simulink model "Shaddad_BMS"  (R2026b)
undefined symbols (not defined in the file): CAN, FD, P, Ts
libraries: simulink x39, stm32blockslib x12, BatteryProtection x7, dspstat3 x7, BatteryEstimators x4, BatteryCurrentManagement x3, eeGeneralControl x2, BatteryBalancing x1, BatterySoeEstimators x1, BatteryPowerEstimators x1, BatteryThermalManagement x1, svdutilitieslib x1
(part 2 of 2)

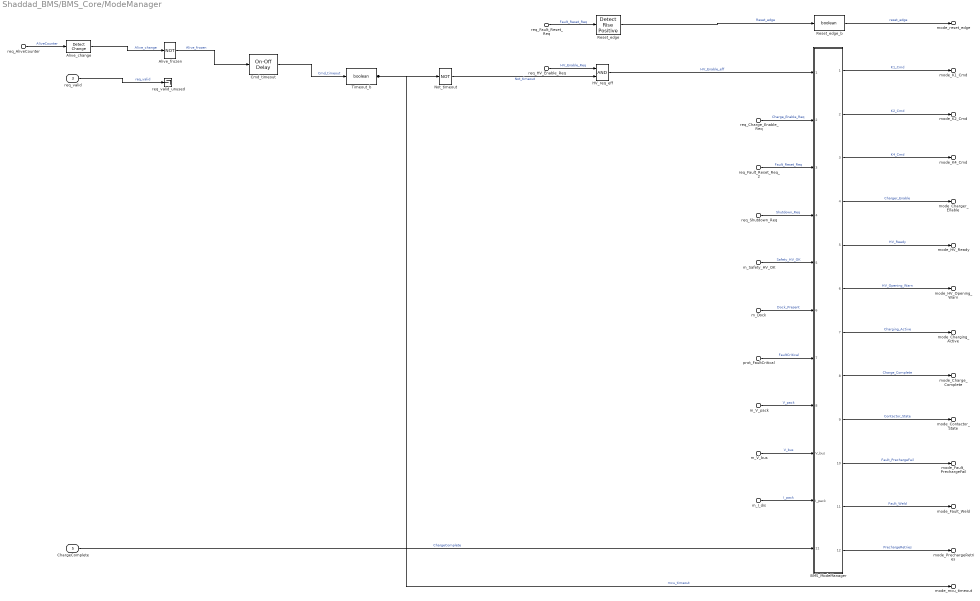
== system Shaddad_BMS/BMS_Core/ModeManager ==
  m_Safety_HV_OK : Inport  PortName=m  Element=Safety_HV_OK
  m_Dock : Inport  PortName=m  Element=Dock
  m_V_pack : Inport  PortName=m  Element=V_pack
  m_V_bus : Inport  PortName=m  Element=V_bus
  m_I_dis : Inport  PortName=m  Element=I_dis
  req_AliveCounter : Inport  Port=2  PortName=req  Element=AliveCounter
  req_HV_Enable_Req : Inport  Port=2  PortName=req  Element=HV_Enable_Req
  req_Fault_Reset_Req : Inport  Port=2  PortName=req  Element=Fault_Reset_Req
  req_Fault_Reset_Req_2 : Inport  Port=2  PortName=req  Element=Fault_Reset_Req
  req_Charge_Enable_Req : Inport  Port=2  PortName=req  Element=Charge_Enable_Req
  req_Shutdown_Req : Inport  Port=2  PortName=req  Element=Shutdown_Req
  req_valid : Inport  Port=3
  prot_FaultCritical : Inport  Port=4  PortName=prot  Element=FaultCritical
  ChargeComplete : Inport  Port=5
  Alive_change : simulink/Logic and Bit Operations/Detect Change  vinit=0  OutDataTypeStr=boolean
  Alive_frozen : Logic  Operator=NOT  AllPortsSameDT=off  OutDataTypeStr=boolean
  BMS_ModeManager : MATLAB Function  TreatAsAtomicUnit=on  mask{prm=P.power.bms.chart}
      mask prompts: prm "Mode manager parameters"
  Cmd_timeout : eeGeneralControl/On-Off Delay  LabelModeActiveChoice=Discrete  Td_on=P.power.bms.mcu_cmd_timeout  Td_off=0  IC=0  Ts=Ts.bms_fast
      settings: LibrarySourceBlock=ee_sl_lib/General Control/On-Off Delay
  HV_req_eff : Logic  AllPortsSameDT=off  OutDataTypeStr=boolean
  Not_timeout : Logic  Operator=NOT  AllPortsSameDT=off  OutDataTypeStr=boolean
  Reset_edge : simulink/Logic and Bit Operations/Detect Rise Positive  vinit=0  OutDataTypeStr=boolean
  Reset_edge_b : DataTypeConversion  OutDataTypeStr=boolean  SaturateOnIntegerOverflow=off  RndMeth=Floor
  Timeout_b : DataTypeConversion  OutDataTypeStr=boolean  SaturateOnIntegerOverflow=off  RndMeth=Floor
  req_valid_unused : Terminator
  mode_mcu_timeout : Outport  PortName=mode  Element=mcu_timeout
  mode_reset_edge : Outport  PortName=mode  Element=reset_edge
  mode_K1_Cmd : Outport  PortName=mode  Element=K1_Cmd
  mode_K2_Cmd : Outport  PortName=mode  Element=K2_Cmd
  mode_K4_Cmd : Outport  PortName=mode  Element=K4_Cmd
  mode_Charger_Enable : Outport  PortName=mode  Element=Charger_Enable
  mode_HV_Ready : Outport  PortName=mode  Element=HV_Ready
  mode_HV_Opening_Warn : Outport  PortName=mode  Element=HV_Opening_Warn
  mode_Charging_Active : Outport  PortName=mode  Element=Charging_Active
  mode_Charge_Complete : Outport  PortName=mode  Element=Charge_Complete
  mode_Contactor_State : Outport  PortName=mode  Element=Contactor_State
  mode_Fault_PrechargeFail : Outport  PortName=mode  Element=Fault_PrechargeFail
  mode_Fault_Weld : Outport  PortName=mode  Element=Fault_Weld
  mode_PrechargeRetries : Outport  PortName=mode  Element=PrechargeRetries
  wires:
  req_AliveCounter/1 -> Alive_change/1  "AliveCounter"
  req_valid/1 -> req_valid_unused/1  "req_valid"
  ChargeComplete/1 -> BMS_ModeManager/11(ChargeComplete)  "ChargeComplete"
  Alive_change/1 -> Alive_frozen/1  "Alive_change"
  Alive_frozen/1 -> Cmd_timeout/1  "Alive_frozen"
  Cmd_timeout/1 -> Timeout_b/1  "Cmd_timeout"
  Timeout_b/1 -> mode_mcu_timeout/1, Not_timeout/1  "mcu_timeout"
  Not_timeout/1 -> HV_req_eff/2  "Not_timeout"
  req_Fault_Reset_Req/1 -> Reset_edge/1  "Fault_Reset_Req"
  req_HV_Enable_Req/1 -> HV_req_eff/1  "HV_Enable_Req"
  HV_req_eff/1 -> BMS_ModeManager/1(HV_Enable_Req)  "HV_Enable_eff"
  Reset_edge/1 -> Reset_edge_b/1  "Reset_edge"
  req_Charge_Enable_Req/1 -> BMS_ModeManager/2(Charge_Enable_Req)  "Charge_Enable_Req"
  req_Fault_Reset_Req_2/1 -> BMS_ModeManager/3(Fault_Reset_Req)  "Fault_Reset_Req"
  req_Shutdown_Req/1 -> BMS_ModeManager/4(Shutdown_Req)  "Shutdown_Req"
  m_Safety_HV_OK/1 -> BMS_ModeManager/5(Safety_OK)  "Safety_HV_OK"
  m_Dock/1 -> BMS_ModeManager/6(Dock_Present)  "Dock_Present"
  prot_FaultCritical/1 -> BMS_ModeManager/7(FaultCritical)  "FaultCritical"
  m_V_pack/1 -> BMS_ModeManager/8(V_pack)  "V_pack"
  m_V_bus/1 -> BMS_ModeManager/9(V_bus)  "V_bus"
  m_I_dis/1 -> BMS_ModeManager/10(I_pack)  "I_pack"
  BMS_ModeManager/1(K1_Cmd) -> mode_K1_Cmd/1  "K1_Cmd"
  BMS_ModeManager/2(K2_Cmd) -> mode_K2_Cmd/1  "K2_Cmd"
  BMS_ModeManager/3(K4_Cmd) -> mode_K4_Cmd/1  "K4_Cmd"
  BMS_ModeManager/4(Charger_Enable) -> mode_Charger_Enable/1  "Charger_Enable"
  BMS_ModeManager/5(HV_Ready) -> mode_HV_Ready/1  "HV_Ready"
  BMS_ModeManager/6(HV_Opening_Warn) -> mode_HV_Opening_Warn/1  "HV_Opening_Warn"
  BMS_ModeManager/7(Charging_Active) -> mode_Charging_Active/1  "Charging_Active"
  BMS_ModeManager/8(Charge_Complete) -> mode_Charge_Complete/1  "Charge_Complete"
  BMS_ModeManager/9(Contactor_State) -> mode_Contactor_State/1  "Contactor_State"
  BMS_ModeManager/10(Fault_PrechargeFail) -> mode_Fault_PrechargeFail/1  "Fault_PrechargeFail"
  BMS_ModeManager/11(Fault_Weld) -> mode_Fault_Weld/1  "Fault_Weld"
  BMS_ModeManager/12(PrechargeRetries) -> mode_PrechargeRetries/1  "PrechargeRetries"
  Reset_edge_b/1 -> mode_reset_edge/1  "reset_edge"

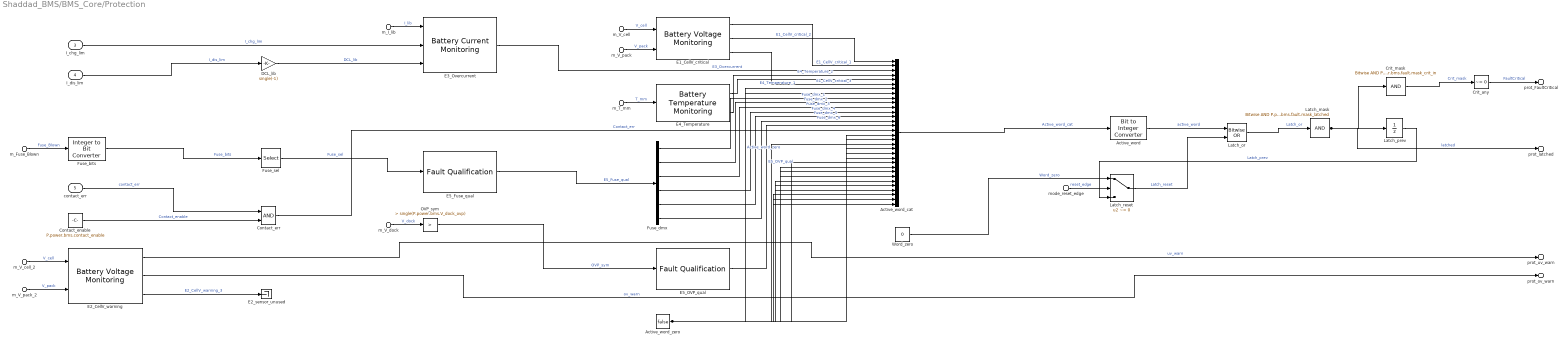
== system Shaddad_BMS/BMS_Core/Protection ==
  m_V_cell : Inport  PortName=m  Element=V_cell
  m_V_cell_2 : Inport  PortName=m  Element=V_cell
  m_V_pack : Inport  PortName=m  Element=V_pack
  m_V_pack_2 : Inport  PortName=m  Element=V_pack
  m_I_lib : Inport  PortName=m  Element=I_lib
  m_T_mm : Inport  PortName=m  Element=T_mm
  m_Fuse_Blown : Inport  PortName=m  Element=Fuse_Blown
  m_V_dock : Inport  PortName=m  Element=V_dock
  mode_reset_edge : Inport  Port=2  PortName=mode  Element=reset_edge
  I_chg_lim : Inport  Port=3
  I_dis_lim : Inport  Port=4
  contact_err : Inport  Port=5
  Active_word : simulink/Logic and Bit Operations/Bit to Integer Converter  nbits=32  bitOrder=LSB first  signedOutputValues=Unsigned  outDtype=uint32  outDtypeSigned=Inherit via internal rule
      settings: LibrarySourceBlock=|
      | commutil2/Bit to Integer
      | Converter
  Active_word_cat : Concatenate  NumInputs=32
  Active_word_zero : Constant  Value=false  OutDataTypeStr=boolean  SampleTime=Ts.bms_fast
  Contact_enable : Constant  Value=P.power.bms.contact_enable  OutDataTypeStr=boolean  SampleTime=Ts.bms_fast
  Contact_err : Logic  AllPortsSameDT=off  OutDataTypeStr=boolean
  Crit_any : simulink/Logic and Bit Operations/Compare To Zero  relop=~=  OutDataTypeStr=boolean
  Crit_mask : simulink/Logic and Bit Operations/Bitwise Operator  logicop=AND  UseBitMask=on  BitMask=P.power.bms.fault.mask_crit_in  BitMaskRealWorld=Stored Integer
  DCL_lib : Gain  Gain=single(-1)
  E1_CellV_critical : BatteryProtection/Battery Voltage Monitoring  UndervoltageLimit=single(P.power.bms.V_uv)  OvervoltageLimit=single(P.power.bms.V_ov)  FaultySensorThreshold=single(P.power.bms.FaultySensorThreshold)  QualTimeUndervoltage=P.power.bms.qual.UV  DisqualTimeUndervoltage=P.power.bms.disqual  QualTimeOvervoltage=P.power.bms.qual.OV  DisqualTimeOvervoltage=P.power.bms.disqual  QualTimeSensorFaulty=P.power.bms.qual.sensor  DisqualTimeSensorFaulty=P.power.bms.disqual  Ts=-1  DataType=single
      settings: LibrarySourceBlock=|
      | batt_sl_lib/Protection/Battery Voltage
      | Monitoring
  E2_CellV_warning : BatteryProtection/Battery Voltage Monitoring  UndervoltageLimit=single(P.power.bms.V_uv_warn)  OvervoltageLimit=single(P.power.bms.V_ov_warn)  FaultySensorThreshold=single(P.power.bms.FaultySensorThreshold)  QualTimeUndervoltage=5  DisqualTimeUndervoltage=5  QualTimeOvervoltage=5  DisqualTimeOvervoltage=5  QualTimeSensorFaulty=5  DisqualTimeSensorFaulty=5  Ts=-1  DataType=single
      settings: LibrarySourceBlock=|
      | batt_sl_lib/Protection/Battery Voltage
      | Monitoring
  E2_sensor_unused : Terminator
  E3_Overcurrent : BatteryProtection/Battery Current Monitoring  ErrorLimit=single(P.power.bms.OC_ErrorLimit)  QualTime=P.power.bms.qual.OC  DisqualTime=P.power.bms.disqual  Ts=-1  DataType=single
      settings: LibrarySourceBlock=|
      | batt_sl_lib/Protection/Battery Current
      | Monitoring
  E4_Temperature : BatteryProtection/Battery Temperature Monitoring  MinMaxFlag=on  UndertemperatureLimit=single(P.power.bms.T_ut)  OvertemperatureLimit=single(P.power.bms.T_ot)  QualTimeUndertemp=P.power.bms.qual.OT  DisqualTimeUndertemp=P.power.bms.disqual  QualTimeOvertemp=P.power.bms.qual.OT  DisqualTimeOvertemp=P.power.bms.disqual  Ts=-1  DataType=single
      settings: LibrarySourceBlock=|
      | batt_sl_lib/Protection/Battery Temperature
      | Monitoring
  E5_Fuse_qual : BatteryProtection/Fault Qualification  QualTime=P.power.bms.qual_aux  DisqualTime=P.power.bms.disqual  Ts=-1
      settings: LibrarySourceBlock=batt_sl_lib/Protection/Fault Qualification
  E5_OVP_qual : BatteryProtection/Fault Qualification  QualTime=P.power.bms.qual_aux  DisqualTime=P.power.bms.disqual  Ts=-1
      settings: LibrarySourceBlock=batt_sl_lib/Protection/Fault Qualification
  Fuse_bits : simulink/Logic and Bit Operations/Integer to Bit Converter  nbits=8  signedInputValues=Unsigned  bitOrder=LSB first  outDtype=boolean
      settings: LibrarySourceBlock=|
      | commutil2/Integer to Bit
      | Converter
  Fuse_dmx : Demux  Outputs=6
  Fuse_sel : Selector  InputPortWidth=8  IndexOptions=Index vector (dialog)  Indices=1:6  OutputSizes=1
  Latch_mask : simulink/Logic and Bit Operations/Bitwise Operator  logicop=AND  UseBitMask=on  BitMask=P.power.bms.fault.mask_latched  BitMaskRealWorld=Stored Integer
  Latch_or : simulink/Logic and Bit Operations/Bitwise Operator  logicop=OR  UseBitMask=off  NumInputPorts=2  BitMask=bin2dec('11011001')  BitMaskRealWorld=Stored Integer
  Latch_prev : UnitDelay  InitialCondition=uint32(0)  SampleTime=Ts.bms_fast
  Latch_reset : Switch  Criteria=u2 ~= 0  SaturateOnIntegerOverflow=off  InputSameDT=off
  OVP_sym : simulink/Logic and Bit Operations/Compare To Constant  relop=>  const=single(P.power.bms.V_dock_ovp)  OutDataTypeStr=boolean
  Word_zero : Constant  Value=0  OutDataTypeStr=uint32  SampleTime=Ts.bms_fast
  prot_uv_warn : Outport  PortName=prot  Element=uv_warn
  prot_ov_warn : Outport  PortName=prot  Element=ov_warn
  prot_latched : Outport  PortName=prot  Element=latched
  prot_FaultCritical : Outport  PortName=prot  Element=FaultCritical
  wires:
  m_Fuse_Blown/1 -> Fuse_bits/1  "Fuse_Blown"
  m_V_cell_2/1 -> E2_CellV_warning/1  "V_cell"
  m_V_pack_2/1 -> E2_CellV_warning/2  "V_pack"
  I_chg_lim/1 -> E3_Overcurrent/2  "I_chg_lim"
  I_dis_lim/1 -> DCL_lib/1  "I_dis_lim"
  contact_err/1 -> Contact_err/1  "contact_err"
  Contact_enable/1 -> Contact_err/2  "Contact_enable"
  Fuse_bits/1 -> Fuse_sel/1  "Fuse_bits"
  E2_CellV_warning/1 -> prot_uv_warn/1  "uv_warn"
  E2_CellV_warning/2 -> prot_ov_warn/1  "ov_warn"
  E2_CellV_warning/3 -> E2_sensor_unused/1  "E2_CellV_warning_3"
  DCL_lib/1 -> E3_Overcurrent/3  "DCL_lib"
  Contact_err/1 -> Active_word_cat/16  "Contact_err"
  Fuse_sel/1 -> E5_Fuse_qual/1  "Fuse_sel"
  m_I_lib/1 -> E3_Overcurrent/1  "I_lib"
  m_V_dock/1 -> OVP_sym/1  "V_dock"
  OVP_sym/1 -> E5_OVP_qual/1  "OVP_sym"
  E3_Overcurrent/1 -> Active_word_cat/3  "E3_Overcurrent"
  E5_Fuse_qual/1 -> Fuse_dmx/1  "E5_Fuse_qual"
  m_V_cell/1 -> E1_CellV_critical/1  "V_cell"
  m_V_pack/1 -> E1_CellV_critical/2  "V_pack"
  m_T_mm/1 -> E4_Temperature/1  "T_mm"
  Fuse_dmx/1 -> Active_word_cat/9  "Fuse_dmx_1"
  Fuse_dmx/2 -> Active_word_cat/10  "Fuse_dmx_2"
  Fuse_dmx/3 -> Active_word_cat/11  "Fuse_dmx_3"
  Fuse_dmx/4 -> Active_word_cat/12  "Fuse_dmx_4"
  Fuse_dmx/5 -> Active_word_cat/13  "Fuse_dmx_5"
  Fuse_dmx/6 -> Active_word_cat/14  "Fuse_dmx_6"
  Active_word_zero/1 -> Active_word_cat/7, Active_word_cat/8, Active_word_cat/17, Active_word_cat/18, Active_word_cat/19, Active_word_cat/20, Active_word_cat/21, Active_word_cat/22, Active_word_cat/23, Active_word_cat/24, Active_word_cat/25, Active_word_cat/26, Active_word_cat/27, Active_word_cat/28, Active_word_cat/29, Active_word_cat/30, Active_word_cat/31, Active_word_cat/32  "Active_word_zero"
  E1_CellV_critical/1 -> Active_word_cat/2  "E1_CellV_critical_1"
  E1_CellV_critical/2 -> Active_word_cat/1  "E1_CellV_critical_2"
  E1_CellV_critical/3 -> Active_word_cat/6  "E1_CellV_critical_3"
  E4_Temperature/1 -> Active_word_cat/5  "E4_Temperature_1"
  E4_Temperature/2 -> Active_word_cat/4  "E4_Temperature_2"
  E5_OVP_qual/1 -> Active_word_cat/15  "E5_OVP_qual"
  Active_word_cat/1 -> Active_word/1  "Active_word_cat"
  Word_zero/1 -> Latch_reset/1  "Word_zero"
  mode_reset_edge/1 -> Latch_reset/2  "reset_edge"
  Latch_reset/1 -> Latch_or/2  "Latch_reset"
  Active_word/1 -> Latch_or/1  "active_word"
  Latch_or/1 -> Latch_mask/1  "Latch_or"
  Latch_mask/1 -> Crit_mask/1, prot_latched/1, Latch_prev/1  "latched"
  Latch_prev/1 -> Latch_reset/3  "Latch_prev"
  Crit_mask/1 -> Crit_any/1  "Crit_mask"
  Crit_any/1 -> prot_FaultCritical/1  "FaultCritical"

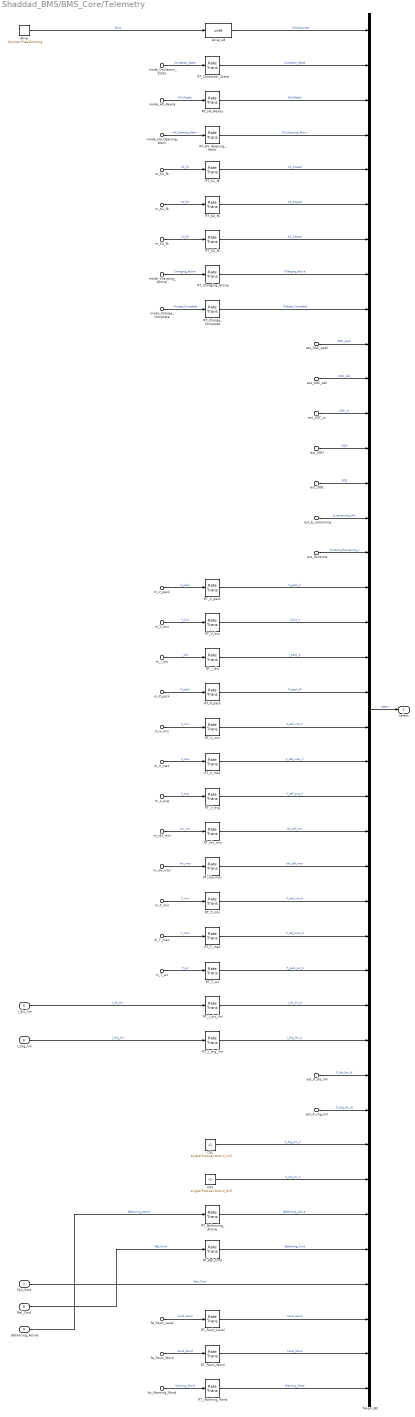
== system Shaddad_BMS/BMS_Core/Telemetry ==
  m_V_pack : Inport  PortName=m  Element=V_pack
  m_V_bus : Inport  PortName=m  Element=V_bus
  m_I_dis : Inport  PortName=m  Element=I_dis
  m_P_pack : Inport  PortName=m  Element=P_pack
  m_V_min : Inport  PortName=m  Element=V_min
  m_V_max : Inport  PortName=m  Element=V_max
  m_V_avg : Inport  PortName=m  Element=V_avg
  m_idx_min : Inport  PortName=m  Element=idx_min
  m_idx_max : Inport  PortName=m  Element=idx_max
  m_T_min : Inport  PortName=m  Element=T_min
  m_T_max : Inport  PortName=m  Element=T_max
  m_T_air : Inport  PortName=m  Element=T_air
  m_K1_fb : Inport  PortName=m  Element=K1_fb
  m_K2_fb : Inport  PortName=m  Element=K2_fb
  m_K4_fb : Inport  PortName=m  Element=K4_fb
  mode_Contactor_State : Inport  Port=2  PortName=mode  Element=Contactor_State
  mode_HV_Ready : Inport  Port=2  PortName=mode  Element=HV_Ready
  mode_HV_Opening_Warn : Inport  Port=2  PortName=mode  Element=HV_Opening_Warn
  mode_Charging_Active : Inport  Port=2  PortName=mode  Element=Charging_Active
  mode_Charge_Complete : Inport  Port=2  PortName=mode  Element=Charge_Complete
  est_SOC_pack : Inport  Port=3  PortName=est  Element=SOC_pack
  est_SOC_cell : Inport  Port=3  PortName=est  Element=SOC_cell
  est_SOC_cc : Inport  Port=3  PortName=est  Element=SOC_cc
  est_SOH : Inport  Port=3  PortName=est  Element=SOH
  est_SOE : Inport  Port=3  PortName=est  Element=SOE
  est_E_remaining : Inport  Port=3  PortName=est  Element=E_remaining
  est_Runtime : Inport  Port=3  PortName=est  Element=Runtime
  est_P_dis_lim : Inport  Port=3  PortName=est  Element=P_dis_lim
  est_P_chg_lim : Inport  Port=3  PortName=est  Element=P_chg_lim
  fw_Fault_Word : Inport  Port=4  PortName=fw  Element=Fault_Word
  fw_Warning_Word : Inport  Port=4  PortName=fw  Element=Warning_Word
  fw_Fault_Level : Inport  Port=4  PortName=fw  Element=Fault_Level
  I_dis_lim : Inport  Port=5
  I_chg_lim : Inport  Port=6
  Fan_Cmd : Inport  Port=7
  Bal_Cmd : Inport  Port=8
  Balancing_Active : Inport  Port=9
  Alive : simulink/Sources/Counter Free-Running  NumBits=8  tsamp=Ts.hk
  Alive_u8 : DataTypeConversion  OutDataTypeStr=uint8  RndMeth=Nearest
  CVL : Constant  Value=single(P.power.bms.V_cvl)  OutDataTypeStr=single  SampleTime=Ts.hk
  DVL : Constant  Value=single(P.power.bms.V_dvl)  OutDataTypeStr=single  SampleTime=Ts.hk
  RT_Bal_Cmd : RateTransition  OutPortSampleTime=Ts.hk
  RT_Balancing_Active : RateTransition  OutPortSampleTime=Ts.hk
  RT_Charge_Complete : RateTransition  OutPortSampleTime=Ts.hk
  RT_Charging_Active : RateTransition  OutPortSampleTime=Ts.hk
  RT_Contactor_State : RateTransition  OutPortSampleTime=Ts.hk
  RT_Fault_Level : RateTransition  OutPortSampleTime=Ts.hk
  RT_Fault_Word : RateTransition  OutPortSampleTime=Ts.hk
  RT_HV_Opening_Warn : RateTransition  OutPortSampleTime=Ts.hk
  RT_HV_Ready : RateTransition  OutPortSampleTime=Ts.hk
  RT_I_chg_lim : RateTransition  OutPortSampleTime=Ts.hk
  RT_I_dis : RateTransition  OutPortSampleTime=Ts.hk
  RT_I_dis_lim : RateTransition  OutPortSampleTime=Ts.hk
  RT_K1_fb : RateTransition  OutPortSampleTime=Ts.hk
  RT_K2_fb : RateTransition  OutPortSampleTime=Ts.hk
  RT_K4_fb : RateTransition  OutPortSampleTime=Ts.hk
  RT_P_pack : RateTransition  OutPortSampleTime=Ts.hk
  RT_T_air : RateTransition  OutPortSampleTime=Ts.hk
  RT_T_max : RateTransition  OutPortSampleTime=Ts.hk
  RT_T_min : RateTransition  OutPortSampleTime=Ts.hk
  RT_V_avg : RateTransition  OutPortSampleTime=Ts.hk
  RT_V_bus : RateTransition  OutPortSampleTime=Ts.hk
  RT_V_max : RateTransition  OutPortSampleTime=Ts.hk
  RT_V_min : RateTransition  OutPortSampleTime=Ts.hk
  RT_V_pack : RateTransition  OutPortSampleTime=Ts.hk
  RT_Warning_Word : RateTransition  OutPortSampleTime=Ts.hk
  RT_idx_max : RateTransition  OutPortSampleTime=Ts.hk
  RT_idx_min : RateTransition  OutPortSampleTime=Ts.hk
  Telem_BC : BusCreator  Inputs=40  OutDataTypeStr=Bus: Bus_BMS_Telemetry  NonVirtualBus=on
      settings: InheritFromInputs=off
  telem : Outport
  wires:
  Alive/1 -> Alive_u8/1  "Alive"
  I_dis_lim/1 -> RT_I_dis_lim/1  "I_dis_lim"
  I_chg_lim/1 -> RT_I_chg_lim/1  "I_chg_lim"
  Fan_Cmd/1 -> Telem_BC/37  "Fan_Cmd"
  Bal_Cmd/1 -> RT_Bal_Cmd/1  "Bal_Cmd"
  Balancing_Active/1 -> RT_Balancing_Active/1  "Balancing_Active"
  mode_Contactor_State/1 -> RT_Contactor_State/1  "Contactor_State"
  mode_HV_Ready/1 -> RT_HV_Ready/1  "HV_Ready"
  mode_HV_Opening_Warn/1 -> RT_HV_Opening_Warn/1  "HV_Opening_Warn"
  m_K1_fb/1 -> RT_K1_fb/1  "K1_fb"
  m_K2_fb/1 -> RT_K2_fb/1  "K2_fb"
  m_K4_fb/1 -> RT_K4_fb/1  "K4_fb"
  mode_Charging_Active/1 -> RT_Charging_Active/1  "Charging_Active"
  mode_Charge_Complete/1 -> RT_Charge_Complete/1  "Charge_Complete"
  m_V_pack/1 -> RT_V_pack/1  "V_pack"
  m_V_bus/1 -> RT_V_bus/1  "V_bus"
  m_I_dis/1 -> RT_I_dis/1  "I_dis"
  m_P_pack/1 -> RT_P_pack/1  "P_pack"
  m_V_min/1 -> RT_V_min/1  "V_min"
  m_V_max/1 -> RT_V_max/1  "V_max"
  m_V_avg/1 -> RT_V_avg/1  "V_avg"
  m_idx_min/1 -> RT_idx_min/1  "idx_min"
  m_idx_max/1 -> RT_idx_max/1  "idx_max"
  m_T_min/1 -> RT_T_min/1  "T_min"
  m_T_max/1 -> RT_T_max/1  "T_max"
  m_T_air/1 -> RT_T_air/1  "T_air"
  fw_Fault_Level/1 -> RT_Fault_Level/1  "Fault_Level"
  fw_Fault_Word/1 -> RT_Fault_Word/1  "Fault_Word"
  fw_Warning_Word/1 -> RT_Warning_Word/1  "Warning_Word"
  CVL/1 -> Telem_BC/33  "V_chg_lim_V"
  DVL/1 -> Telem_BC/34  "V_dis_lim_V"
  RT_Contactor_State/1 -> Telem_BC/2  "Contactor_State"
  RT_HV_Ready/1 -> Telem_BC/3  "HV_Ready"
  RT_HV_Opening_Warn/1 -> Telem_BC/4  "HV_Opening_Warn"
  RT_K1_fb/1 -> Telem_BC/5  "K1_Closed"
  RT_K2_fb/1 -> Telem_BC/6  "K2_Closed"
  RT_K4_fb/1 -> Telem_BC/7  "K4_Closed"
  RT_Charging_Active/1 -> Telem_BC/8  "Charging_Active"
  RT_Charge_Complete/1 -> Telem_BC/9  "Charge_Complete"
  RT_V_pack/1 -> Telem_BC/17  "V_pack_V"
  RT_V_bus/1 -> Telem_BC/18  "V_bus_V"
  RT_I_dis/1 -> Telem_BC/19  "I_pack_A"
  RT_P_pack/1 -> Telem_BC/20  "P_pack_W"
  RT_V_min/1 -> Telem_BC/21  "V_cell_min_V"
  RT_V_max/1 -> Telem_BC/22  "V_cell_max_V"
  RT_V_avg/1 -> Telem_BC/23  "V_cell_avg_V"
  RT_idx_min/1 -> Telem_BC/24  "idx_cell_min"
  RT_idx_max/1 -> Telem_BC/25  "idx_cell_max"
  RT_T_min/1 -> Telem_BC/26  "T_cell_min_K"
  RT_T_max/1 -> Telem_BC/27  "T_cell_max_K"
  RT_T_air/1 -> Telem_BC/28  "T_pack_air_K"
  RT_I_dis_lim/1 -> Telem_BC/29  "I_dis_lim_A"
  RT_I_chg_lim/1 -> Telem_BC/30  "I_chg_lim_A"
  RT_Balancing_Active/1 -> Telem_BC/35  "Balancing_Active"
  RT_Bal_Cmd/1 -> Telem_BC/36  "Balancing_Cmd"
  RT_Fault_Level/1 -> Telem_BC/38  "Fault_Level"
  RT_Fault_Word/1 -> Telem_BC/39  "Fault_Word"
  RT_Warning_Word/1 -> Telem_BC/40  "Warning_Word"
  Alive_u8/1 -> Telem_BC/1  "AliveCounter"
  est_SOC_pack/1 -> Telem_BC/10  "SOC_pack"
  est_SOC_cell/1 -> Telem_BC/11  "SOC_cell"
  est_SOC_cc/1 -> Telem_BC/12  "SOC_cc"
  est_SOH/1 -> Telem_BC/13  "SOH"
  est_SOE/1 -> Telem_BC/14  "SOE"
  est_E_remaining/1 -> Telem_BC/15  "E_remaining_Wh"
  est_Runtime/1 -> Telem_BC/16  "Runtime_Remaining_s"
  est_P_dis_lim/1 -> Telem_BC/31  "P_dis_lim_W"
  est_P_chg_lim/1 -> Telem_BC/32  "P_chg_lim_W"
  Telem_BC/1 -> telem/1  "telem"

== system Shaddad_BMS/BMS_Core/Thermal ==
  m_T_amb : Inport  PortName=m  Element=T_amb
  m_T_air : Inport  PortName=m  Element=T_air
  m_T_mm : Inport  PortName=m  Element=T_mm
  m_T_max : Inport  PortName=m  Element=T_max
  Cells_hotter : simulink/Logic and Bit Operations/Compare To Constant  relop=>  const=single(-P.power.bms.fan.dT_amb)  OutDataTypeStr=boolean
  E17_Fan_control : BatteryThermalManagement/Battery Coolant Control  MinMaxFlag=on  ControlStrategy=ON-OFF control  TempOn=single(P.power.thermal.TempOn)  TempOff=single(P.power.thermal.TempOff)  c=single(0.1)  FlowRateStep=single(0.2)  DataType=single
      settings: LibrarySourceBlock=batt_sl_lib/Thermal Management/Battery Coolant Control
  Fan_and : Logic  AllPortsSameDT=off  OutDataTypeStr=boolean
  Fan_on : simulink/Logic and Bit Operations/Compare To Zero  relop=>  OutDataTypeStr=boolean
  Fan_or : Logic  Operator=OR  AllPortsSameDT=off  OutDataTypeStr=boolean
  Fan_single : DataTypeConversion  OutDataTypeStr=single  SaturateOnIntegerOverflow=off  RndMeth=Floor
  FlowT_unused : Terminator
  Forced : simulink/Logic and Bit Operations/Compare To Constant  relop=>  const=single(P.power.bms.fan.T_force)  OutDataTypeStr=boolean
  RT_T_air : RateTransition  OutPortSampleTime=Ts.bms_slow
  RT_T_amb : RateTransition  OutPortSampleTime=Ts.bms_slow
  RT_T_max : RateTransition  OutPortSampleTime=Ts.bms_slow
  RT_T_mm : RateTransition  OutPortSampleTime=Ts.bms_slow
  dT_amb : Sum  Inputs=+-
  Fan_Cmd : Outport
  wires:
  m_T_air/1 -> RT_T_air/1  "T_air"
  m_T_mm/1 -> RT_T_mm/1  "T_mm"
  m_T_amb/1 -> RT_T_amb/1  "T_amb"
  m_T_max/1 -> RT_T_max/1  "T_max"
  RT_T_air/1 -> E17_Fan_control/2  "RT_T_air"
  RT_T_mm/1 -> E17_Fan_control/3  "RT_T_mm"
  RT_T_amb/1 -> E17_Fan_control/1, dT_amb/2  "RT_T_amb"
  RT_T_max/1 -> Forced/1, dT_amb/1  "RT_T_max"
  dT_amb/1 -> Cells_hotter/1  "dT_amb"
  E17_Fan_control/1 -> Fan_on/1  "E17_Fan_control_1"
  E17_Fan_control/2 -> FlowT_unused/1  "E17_Fan_control_2"
  Fan_on/1 -> Fan_and/1  "Fan_on"
  Cells_hotter/1 -> Fan_and/2  "Cells_hotter"
  Fan_and/1 -> Fan_or/1  "Fan_and"
  Forced/1 -> Fan_or/2  "Forced"
  Fan_or/1 -> Fan_single/1  "Fan_or"
  Fan_single/1 -> Fan_Cmd/1  "Fan_Cmd"

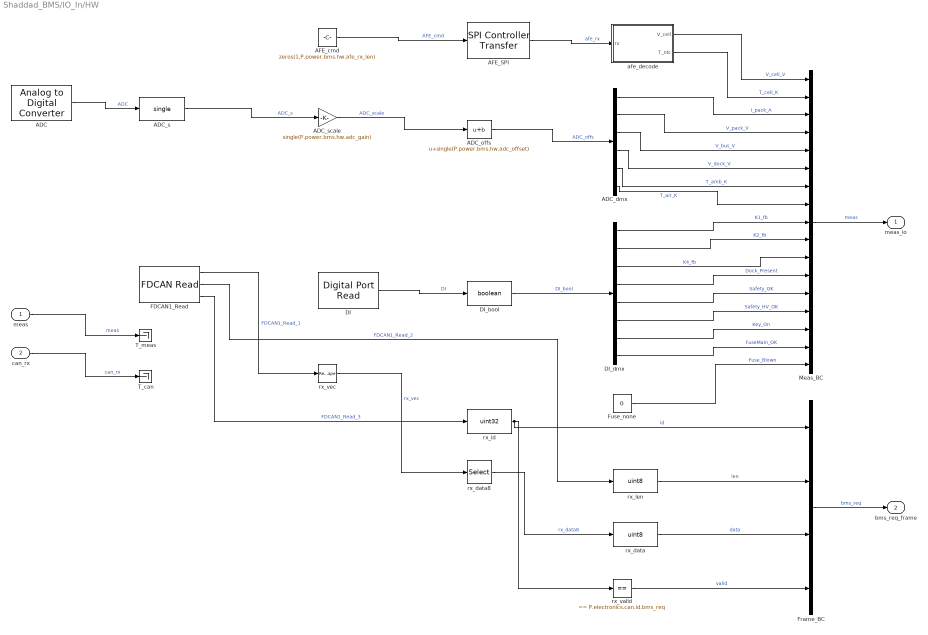
== system Shaddad_BMS/IO_In/HW ==
  meas : Inport
  can_rx : Inport  Port=2
  ADC : stm32blockslib/Analog to Digital Converter  ADCModule=ADC1  ConversionGroup=Regular  TriggerMode=Trigger and read  NumberOfConversions=1  EnableBufferConv=off  BufferLength=1  OutputStatus=off  SampleTime=-1
  ADC_dmx : Demux  Outputs=6
  ADC_offs : Bias  Bias=single(P.power.bms.hw.adc_offset)  SaturateOnIntegerOverflow=off
  ADC_s : DataTypeConversion  OutDataTypeStr=single  SaturateOnIntegerOverflow=off  RndMeth=Floor
  ADC_scale : Gain  Gain=single(P.power.bms.hw.adc_gain)
  AFE_SPI : stm32blockslib/SPI Controller Transfer  SPIModuleSelect=SPI1  ClockPolarity=Low  ClockPhase=1 Edge  SPIModule=uint32(0)  Mode=Master  BusSpeed=uint32(1000000)  FirstBitToTransfer=Most significant bit (MSB)  ClockMode=0  BlockFunction=Transfer  EnableRegisterAddress=on  RegisterAddress=0  OutputDataType=uint8  OutputDataLength=1  OutputStatus=off  BlockingMode=off  Timeout=0.001  DataBits=8  UseCustomSSPin=Provided by the SPI peripheral  ActiveLowSSPin=Active low  Port_Select=GPIOA  Pin=0
  AFE_cmd : Constant  Value=zeros(1,P.power.bms.hw.afe_rx_len)  OutDataTypeStr=uint8  SampleTime=Ts.bms_fast
  DI : stm32blockslib/Digital Port Read  PortName=GPIOC  PinNumber=[4:11]  ReadOperation=on  IOAsArray=on  SampleTime=Ts.bms_fast
  DI_bool : DataTypeConversion  OutDataTypeStr=boolean  SaturateOnIntegerOverflow=off  RndMeth=Floor
  DI_dmx : Demux  Outputs=8
  FDCAN1_Read : stm32blockslib/FDCAN Read  FDCANModule=FDCAN1  BlockMode=Receive  OperationReadMode=Data  OperationWriteMode=Data  ReadSource=FIFO 0  BufferNumber=0  OutputTypeReadMode=Unpacked  DataFormatWriteMode=Raw data  CANFrameType=CAN-FD  IdentifierTypeVia=Dialog  IdentifierType=Standard (11-bit identifier)  IdentifierVia=Inport  Identifier=100  DataLengthVia=Inport  DataLength=64  OutputIdType=off  IsBitRateSwitchingEnabled=off  TransmitRemoteFrame=off  OutputFrameType=off  OutputBRS=off  OutputRemoteFrame=off  OutputTxFifoLevel=off  OutputRxFifoLevel=off  OutputStatus=off  Timeout=0.001  SampleTime=Ts.can_slow
  Frame_BC : BusCreator  Inputs=4  OutDataTypeStr=Bus: Bus_CanFrame8  NonVirtualBus=on
      settings: InheritFromInputs=off
  Fuse_none : Constant  Value=0  OutDataTypeStr=uint8  SampleTime=Ts.bms_fast
  Meas_BC : BusCreator  Inputs=17  OutDataTypeStr=Bus: Bus_BMS_Meas  NonVirtualBus=on
      settings: InheritFromInputs=off
  T_can : Terminator
  T_meas : Terminator
  afe_decode : Subsystem
  rx_data : DataTypeConversion  OutDataTypeStr=uint8  SaturateOnIntegerOverflow=off  RndMeth=Floor
  rx_data8 : Selector  IndexOptions=Index vector (dialog)  Indices=1:8  OutputSizes=1
  rx_id : DataTypeConversion  OutDataTypeStr=uint32  SaturateOnIntegerOverflow=off  RndMeth=Floor
  rx_len : DataTypeConversion  OutDataTypeStr=uint8  SaturateOnIntegerOverflow=off  RndMeth=Floor
  rx_valid : simulink/Logic and Bit Operations/Compare To Constant  relop===  const=P.electronics.can.id.bms_req  OutDataTypeStr=boolean
  rx_vec : Reshape
  meas_io : Outport
  bms_req_frame : Outport  Port=2
  wires:
  meas/1 -> T_meas/1  "meas"
  can_rx/1 -> T_can/1  "can_rx"
  ADC/1 -> ADC_s/1  "ADC"
  ADC_s/1 -> ADC_scale/1  "ADC_s"
  FDCAN1_Read/1 -> rx_vec/1  "FDCAN1_Read_1"
  FDCAN1_Read/2 -> rx_len/1  "FDCAN1_Read_2"
  FDCAN1_Read/3 -> rx_id/1  "FDCAN1_Read_3"
  AFE_cmd/1 -> AFE_SPI/1  "AFE_cmd"
  ADC_scale/1 -> ADC_offs/1  "ADC_scale"
  rx_vec/1 -> rx_data8/1  "rx_vec"
  DI/1 -> DI_bool/1  "DI"
  ADC_offs/1 -> ADC_dmx/1  "ADC_offs"
  rx_data8/1 -> rx_data/1  "rx_data8"
  DI_bool/1 -> DI_dmx/1  "DI_bool"
  rx_id/1 -> rx_valid/1, Frame_BC/1  "id"
  AFE_SPI/1 -> afe_decode/1(rx)  "afe_rx"
  ADC_dmx/1 -> Meas_BC/3  "I_pack_A"
  ADC_dmx/2 -> Meas_BC/4  "V_pack_V"
  ADC_dmx/3 -> Meas_BC/5  "V_bus_V"
  ADC_dmx/4 -> Meas_BC/6  "V_dock_V"
  ADC_dmx/5 -> Meas_BC/7  "T_amb_K"
  ADC_dmx/6 -> Meas_BC/8  "T_air_K"
  DI_dmx/1 -> Meas_BC/9  "K1_fb"
  DI_dmx/2 -> Meas_BC/10  "K2_fb"
  DI_dmx/3 -> Meas_BC/11  "K4_fb"
  DI_dmx/4 -> Meas_BC/12  "Dock_Present"
  DI_dmx/5 -> Meas_BC/13  "Safety_OK"
  DI_dmx/6 -> Meas_BC/14  "Safety_HV_OK"
  DI_dmx/7 -> Meas_BC/15  "Key_On"
  DI_dmx/8 -> Meas_BC/16  "FuseMain_OK"
  Fuse_none/1 -> Meas_BC/17  "Fuse_Blown"
  rx_valid/1 -> Frame_BC/4  "valid"
  rx_len/1 -> Frame_BC/2  "len"
  rx_data/1 -> Frame_BC/3  "data"
  afe_decode/1(V_cell) -> Meas_BC/1  "V_cell_V"
  afe_decode/2(T_ntc) -> Meas_BC/2  "T_cell_K"
  Meas_BC/1 -> meas_io/1  "meas"
  Frame_BC/1 -> bms_req_frame/1  "bms_req"

== system Shaddad_BMS/IO_In/SIM ==
  meas : Inport  OutDataTypeStr=Bus: Bus_BMS_Meas
  can_rx : Inport  Port=2  OutDataTypeStr=Bus: Bus_Can1_McuSlow
  Sel_req : BusSelector  OutputSignals=bms_req
  meas_io : Outport
  bms_req_frame : Outport  Port=2
  wires:
  meas/1 -> meas_io/1  "meas"
  can_rx/1 -> Sel_req/1  "can_rx"
  Sel_req/1 -> bms_req_frame/1  "<bms_req>"

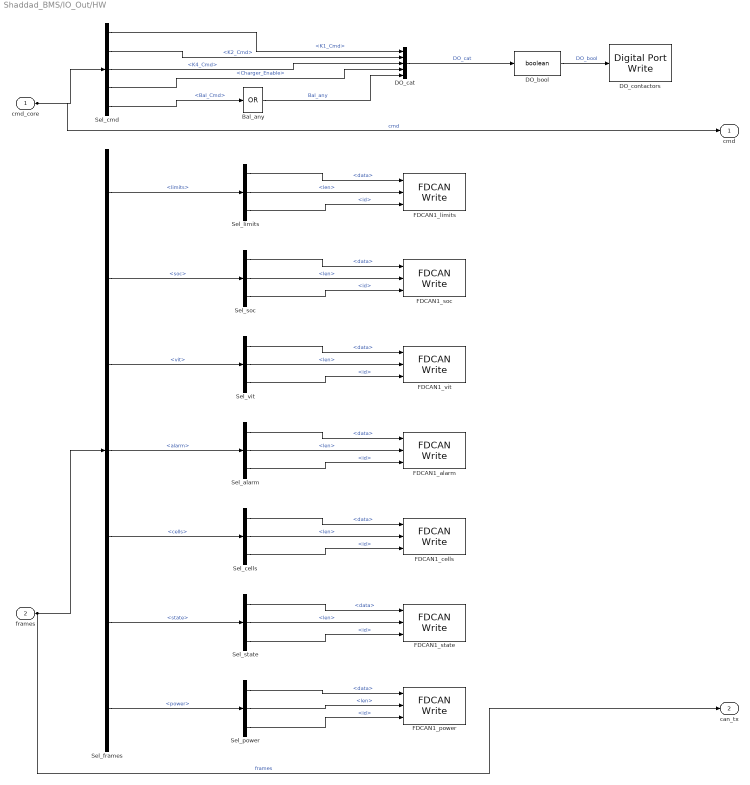
== system Shaddad_BMS/IO_Out/HW ==
  cmd_core : Inport  OutDataTypeStr=Bus: Bus_BMS_Cmd
  frames : Inport  Port=2  OutDataTypeStr=Bus: Bus_Can1_Bms
  Bal_any : Logic  Operator=OR  Inputs=1  AllPortsSameDT=off  OutDataTypeStr=boolean
  DO_bool : DataTypeConversion  OutDataTypeStr=boolean  SaturateOnIntegerOverflow=off  RndMeth=Floor
  DO_cat : Concatenate  NumInputs=5
  DO_contactors : stm32blockslib/Digital Port Write  PortName=GPIOB  PinNumber=[4 5 6 7 10]  ReadOperation=off  IOAsArray=on  SampleTime=-1
  FDCAN1_alarm : stm32blockslib/FDCAN Write  FDCANModule=FDCAN1  BlockMode=Transmit  OperationReadMode=Data  OperationWriteMode=Data  ReadSource=FIFO 0  BufferNumber=0  OutputTypeReadMode=Unpacked  DataFormatWriteMode=Raw data  CANFrameType=CAN  IdentifierTypeVia=Dialog  IdentifierType=Standard (11-bit identifier)  IdentifierVia=Inport  Identifier=100  DataLengthVia=Inport  DataLength=8  OutputIdType=off  IsBitRateSwitchingEnabled=off  TransmitRemoteFrame=off  OutputFrameType=off  OutputBRS=off  OutputRemoteFrame=off  OutputTxFifoLevel=off  OutputRxFifoLevel=off  OutputStatus=off  Timeout=0.001  SampleTime=-1
  FDCAN1_cells : stm32blockslib/FDCAN Write  FDCANModule=FDCAN1  BlockMode=Transmit  OperationReadMode=Data  OperationWriteMode=Data  ReadSource=FIFO 0  BufferNumber=0  OutputTypeReadMode=Unpacked  DataFormatWriteMode=Raw data  CANFrameType=CAN  IdentifierTypeVia=Dialog  IdentifierType=Standard (11-bit identifier)  IdentifierVia=Inport  Identifier=100  DataLengthVia=Inport  DataLength=8  OutputIdType=off  IsBitRateSwitchingEnabled=off  TransmitRemoteFrame=off  OutputFrameType=off  OutputBRS=off  OutputRemoteFrame=off  OutputTxFifoLevel=off  OutputRxFifoLevel=off  OutputStatus=off  Timeout=0.001  SampleTime=-1
  FDCAN1_limits : stm32blockslib/FDCAN Write  FDCANModule=FDCAN1  BlockMode=Transmit  OperationReadMode=Data  OperationWriteMode=Data  ReadSource=FIFO 0  BufferNumber=0  OutputTypeReadMode=Unpacked  DataFormatWriteMode=Raw data  CANFrameType=CAN  IdentifierTypeVia=Dialog  IdentifierType=Standard (11-bit identifier)  IdentifierVia=Inport  Identifier=100  DataLengthVia=Inport  DataLength=8  OutputIdType=off  IsBitRateSwitchingEnabled=off  TransmitRemoteFrame=off  OutputFrameType=off  OutputBRS=off  OutputRemoteFrame=off  OutputTxFifoLevel=off  OutputRxFifoLevel=off  OutputStatus=off  Timeout=0.001  SampleTime=-1
  FDCAN1_power : stm32blockslib/FDCAN Write  FDCANModule=FDCAN1  BlockMode=Transmit  OperationReadMode=Data  OperationWriteMode=Data  ReadSource=FIFO 0  BufferNumber=0  OutputTypeReadMode=Unpacked  DataFormatWriteMode=Raw data  CANFrameType=CAN  IdentifierTypeVia=Dialog  IdentifierType=Standard (11-bit identifier)  IdentifierVia=Inport  Identifier=100  DataLengthVia=Inport  DataLength=8  OutputIdType=off  IsBitRateSwitchingEnabled=off  TransmitRemoteFrame=off  OutputFrameType=off  OutputBRS=off  OutputRemoteFrame=off  OutputTxFifoLevel=off  OutputRxFifoLevel=off  OutputStatus=off  Timeout=0.001  SampleTime=-1
  FDCAN1_soc : stm32blockslib/FDCAN Write  FDCANModule=FDCAN1  BlockMode=Transmit  OperationReadMode=Data  OperationWriteMode=Data  ReadSource=FIFO 0  BufferNumber=0  OutputTypeReadMode=Unpacked  DataFormatWriteMode=Raw data  CANFrameType=CAN  IdentifierTypeVia=Dialog  IdentifierType=Standard (11-bit identifier)  IdentifierVia=Inport  Identifier=100  DataLengthVia=Inport  DataLength=8  OutputIdType=off  IsBitRateSwitchingEnabled=off  TransmitRemoteFrame=off  OutputFrameType=off  OutputBRS=off  OutputRemoteFrame=off  OutputTxFifoLevel=off  OutputRxFifoLevel=off  OutputStatus=off  Timeout=0.001  SampleTime=-1
  FDCAN1_state : stm32blockslib/FDCAN Write  FDCANModule=FDCAN1  BlockMode=Transmit  OperationReadMode=Data  OperationWriteMode=Data  ReadSource=FIFO 0  BufferNumber=0  OutputTypeReadMode=Unpacked  DataFormatWriteMode=Raw data  CANFrameType=CAN  IdentifierTypeVia=Dialog  IdentifierType=Standard (11-bit identifier)  IdentifierVia=Inport  Identifier=100  DataLengthVia=Inport  DataLength=8  OutputIdType=off  IsBitRateSwitchingEnabled=off  TransmitRemoteFrame=off  OutputFrameType=off  OutputBRS=off  OutputRemoteFrame=off  OutputTxFifoLevel=off  OutputRxFifoLevel=off  OutputStatus=off  Timeout=0.001  SampleTime=-1
  FDCAN1_vit : stm32blockslib/FDCAN Write  FDCANModule=FDCAN1  BlockMode=Transmit  OperationReadMode=Data  OperationWriteMode=Data  ReadSource=FIFO 0  BufferNumber=0  OutputTypeReadMode=Unpacked  DataFormatWriteMode=Raw data  CANFrameType=CAN  IdentifierTypeVia=Dialog  IdentifierType=Standard (11-bit identifier)  IdentifierVia=Inport  Identifier=100  DataLengthVia=Inport  DataLength=8  OutputIdType=off  IsBitRateSwitchingEnabled=off  TransmitRemoteFrame=off  OutputFrameType=off  OutputBRS=off  OutputRemoteFrame=off  OutputTxFifoLevel=off  OutputRxFifoLevel=off  OutputStatus=off  Timeout=0.001  SampleTime=-1
  Sel_alarm : BusSelector  OutputSignals=data,len,id
  Sel_cells : BusSelector  OutputSignals=data,len,id
  Sel_cmd : BusSelector  OutputSignals=K1_Cmd,K2_Cmd,K4_Cmd,Charger_Enable,Bal_Cmd
  Sel_frames : BusSelector  OutputSignals=limits,soc,vit,alarm,cells,state,power
  Sel_limits : BusSelector  OutputSignals=data,len,id
  Sel_power : BusSelector  OutputSignals=data,len,id
  Sel_soc : BusSelector  OutputSignals=data,len,id
  Sel_state : BusSelector  OutputSignals=data,len,id
  Sel_vit : BusSelector  OutputSignals=data,len,id
  cmd : Outport
  can_tx : Outport  Port=2
  wires:
  cmd_core/1 -> Sel_cmd/1, cmd/1  "cmd"
  frames/1 -> Sel_frames/1, can_tx/1  "frames"
  Sel_cmd/1 -> DO_cat/1  "<K1_Cmd>"
  Sel_cmd/2 -> DO_cat/2  "<K2_Cmd>"
  Sel_cmd/3 -> DO_cat/3  "<K4_Cmd>"
  Sel_cmd/4 -> DO_cat/4  "<Charger_Enable>"
  Sel_cmd/5 -> Bal_any/1  "<Bal_Cmd>"
  Sel_frames/1 -> Sel_limits/1  "<limits>"
  Sel_frames/2 -> Sel_soc/1  "<soc>"
  Sel_frames/3 -> Sel_vit/1  "<vit>"
  Sel_frames/4 -> Sel_alarm/1  "<alarm>"
  Sel_frames/5 -> Sel_cells/1  "<cells>"
  Sel_frames/6 -> Sel_state/1  "<state>"
  Sel_frames/7 -> Sel_power/1  "<power>"
  Sel_limits/1 -> FDCAN1_limits/1  "<data>"
  Sel_limits/2 -> FDCAN1_limits/2  "<len>"
  Sel_limits/3 -> FDCAN1_limits/3  "<id>"
  Sel_soc/1 -> FDCAN1_soc/1  "<data>"
  Sel_soc/2 -> FDCAN1_soc/2  "<len>"
  Sel_soc/3 -> FDCAN1_soc/3  "<id>"
  Sel_vit/1 -> FDCAN1_vit/1  "<data>"
  Sel_vit/2 -> FDCAN1_vit/2  "<len>"
  Sel_vit/3 -> FDCAN1_vit/3  "<id>"
  Sel_alarm/1 -> FDCAN1_alarm/1  "<data>"
  Sel_alarm/2 -> FDCAN1_alarm/2  "<len>"
  Sel_alarm/3 -> FDCAN1_alarm/3  "<id>"
  Sel_cells/1 -> FDCAN1_cells/1  "<data>"
  Sel_cells/2 -> FDCAN1_cells/2  "<len>"
  Sel_cells/3 -> FDCAN1_cells/3  "<id>"
  Sel_state/1 -> FDCAN1_state/1  "<data>"
  Sel_state/2 -> FDCAN1_state/2  "<len>"
  Sel_state/3 -> FDCAN1_state/3  "<id>"
  Sel_power/1 -> FDCAN1_power/1  "<data>"
  Sel_power/2 -> FDCAN1_power/2  "<len>"
  Sel_power/3 -> FDCAN1_power/3  "<id>"
  Bal_any/1 -> DO_cat/5  "Bal_any"
  DO_cat/1 -> DO_bool/1  "DO_cat"
  DO_bool/1 -> DO_contactors/1  "DO_bool"

== system Shaddad_BMS/IO_Out/SIM ==
  cmd_core : Inport
  frames : Inport  Port=2
  cmd : Outport
  can_tx : Outport  Port=2
  wires:
  cmd_core/1 -> cmd/1  "cmd"
  frames/1 -> can_tx/1  "can_tx"

== system Shaddad_BMS/IO_In/HW/afe_decode ==
  rx : Inport
  NTC_lut : Lookup_n-D  NumberOfTableDimensions=1  BreakpointsForDimension1=single(P.power.bms.hw.ntc_counts)  Table=single(P.power.bms.hw.ntc_K)  ExtrapMethod=Clip  InternalRulePriority=Speed  RndMeth=Simplest
  N_s : DataTypeConversion  OutDataTypeStr=single  SaturateOnIntegerOverflow=off  RndMeth=Floor
  Regs : svdutilitieslib/Byte Unpack  dimensions={13,13}  datatypes={'uint16','uint16'}  byteAlign=1  blockPlatform=arduinoert
      settings: LibrarySourceBlock=mcblib/Signal Management/Byte Unpack
  V_lsb : Gain  Gain=single(P.power.bms.hw.afe_lsb_V)
  V_s : DataTypeConversion  OutDataTypeStr=single  SaturateOnIntegerOverflow=off  RndMeth=Floor
  rx_u8 : DataTypeConversion  OutDataTypeStr=uint8  SaturateOnIntegerOverflow=off  RndMeth=Floor
  V_cell : Outport
  T_ntc : Outport  Port=2
  wires:
  rx/1 -> rx_u8/1  "rx"
  rx_u8/1 -> Regs/1  "rx_u8"
  Regs/1 -> V_s/1  "Regs_1"
  Regs/2 -> N_s/1  "Regs_2"
  V_s/1 -> V_lsb/1  "V_s"
  N_s/1 -> NTC_lut/1  "N_s"
  V_lsb/1 -> V_cell/1  "V_cell"
  NTC_lut/1 -> T_ntc/1  "T_ntc"

== matlab function Shaddad_BMS/BMS_Core/ModeManager/BMS_ModeManager ==
  settings: updateMethod=DISCRETE  sampleTime=Ts.bms_fast  description=BMS mode manager (docs/specs/power.md 4.1), body bms_mode_manager.m; Stateflow not installed (D1).
  data: HV_Enable_Req input; K1_Cmd output; Charge_Enable_Req input; Fault_Reset_Req input; Shutdown_Req input; Safety_OK input; Dock_Present input; FaultCritical input; V_pack input; V_bus input; I_pack input; ChargeComplete input; K2_Cmd output; K4_Cmd output; Charger_Enable output; HV_Ready output; HV_Opening_Warn output; Charging_Active output; Charge_Complete output; Contactor_State output; Fault_PrechargeFail output; Fault_Weld output; PrechargeRetries output; prm parameter
function [K1_Cmd, K2_Cmd, K4_Cmd, Charger_Enable, HV_Ready, HV_Opening_Warn, Charging_Active, Charge_Complete, Contactor_State, Fault_PrechargeFail, Fault_Weld, PrechargeRetries] = fcn(HV_Enable_Req, Charge_Enable_Req, Fault_Reset_Req, Shutdown_Req, Safety_OK, Dock_Present, FaultCritical, V_pack, V_bus, I_pack, ChargeComplete, prm)
%#codegen
[K1_Cmd, K2_Cmd, K4_Cmd, Charger_Enable, HV_Ready, HV_Opening_Warn, Charging_Active, Charge_Complete, Contactor_State, Fault_PrechargeFail, Fault_Weld, PrechargeRetries] = bms_mode_manager(HV_Enable_Req, Charge_Enable_Req, Fault_Reset_Req, Shutdown_Req, Safety_OK, Dock_Present, FaultCritical, V_pack, V_bus, I_pack, ChargeComplete, prm);
